simulink subsystem "Subsys_GFolConv_OuterCtrl_MatchCtrl"  (R2023b)
settings: Solver=VariableStepAuto  StartTime=0.0  StopTime=10.0  RelTol=1e-3
model mask{S_n=S_n, P_binst=P_binst, f_n=f_n, Q_ctrl_mode_m=Matching_Control_Q_ctrl_mode, T_PT1_Q_m=Matching_Control_T_PT1_Q, uq0ref_m=Matching_Control_QV_uq0ref, qmax_m=Matching_Control_QV_qmax, umax_m=Matching_Control_QV_umax, deadband_m=Matching_Control_QV_deadband, p_pu_m=Matching_Control_QP_P, q_pu_m=Matching_Control_QP_Q, p1_m=Matching_Control_QVDB_P1, p2_m=Matching_Control_QVDB_P2, p3_m=Matching_Control_QVDB_P3, p4_m=Matching_Control_QVDB_P4, cosphi_ref_m=Matching_Control_cosphi_ref, Q_direction_m=Matching_Control_cosphi_direction, T_s_ctrl=T_s_ctrl, datatype=datatype, K_matching=K_Matching_m, plant_ref=Plant_Ref, plant_model=Plant_Model, luenberger=Luenberger, Ts_matching=Ts_Matching_m}
  mask prompts: S_n "Nominal apparent power [VA]"; P_binst "Installed active power [W]"; f_n "Nominal frequency [Hz]"; Q_ctrl_mode_m "Q-control mode (1 = Q(V), 2 = Q(P), 3 = Q(V) with deadband, 4 = cosphi)"; T_PT1_Q_m "Time constant of reactive power PT1 delay [s]"; uq0ref_m "U_Q0ref [pu]"; qmax_m "|Q_max| [pu]"; umax_m "U_max [pu]"; deadband_m "Voltage deadband [+-%]"; p_pu_m "P_grid points [pu]"; q_pu_m "Q_grid points [pu]"; p1_m "P1 [V_grid, Q_grid] [pu]"; p2_m "P2 [V_grid, Q_grid] [pu]"; p3_m "P3 [V_grid, Q_grid] [pu]"; p4_m "P4 [V_grid, Q_grid] [pu]"; cosphi_ref_m "cos(phi)"; Q_direction_m "Reactive power flow direction (1 =ind. Q injection, 0 = ind. Q consumption)"; T_s_ctrl "Controller sample time [s]"; datatype "Signal data type"; K_matching "Gain Matching Control"; plant_ref "Reference model"; plant_model "Plant model"; luenberger "Luenberger observer"; Ts_matching "Time constant Matching Control"
undefined symbols (not defined in the file): DiscIntNeverNeededParam
libraries: simulink x5, spsSampleandHoldLib x2, cstblocks x2, dspswit3 x1
settings Model: Creator=j.jansen  LastModifiedBy=a.och
settings RTWCC: GPUComputeCapability=5.0

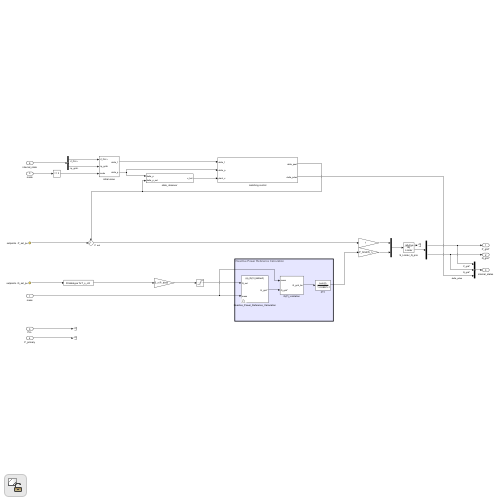
[thumbnail: Simulink's stored preview of the top-level diagram]
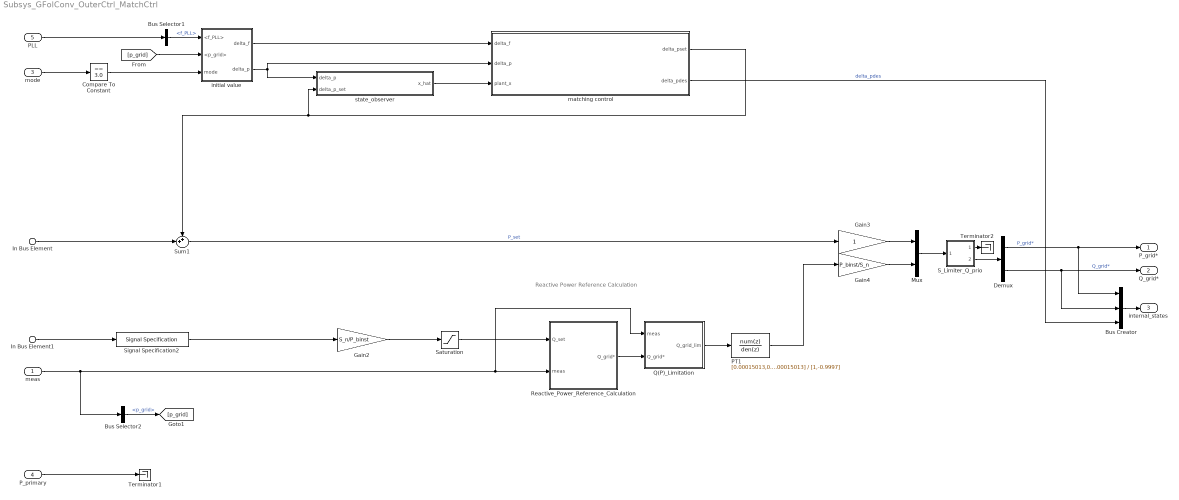
== system Subsys_GFolConv_OuterCtrl_MatchCtrl ==
  note: Reactive Power Reference Calculation
  meas : Inport
  In Bus Element : Inport  Port=2  PortName=setpoints  Element=P_set_pu
  In Bus Element1 : Inport  Port=2  PortName=setpoints  Element=Q_set_pu
  mode : Inport  Port=3
  P_primary : Inport  Port=4
  PLL : Inport  Port=5
  Bus Creator : BusCreator  Inputs=3
  Bus Selector1 : BusSelector  OutputSignals=f_PLL
  Bus Selector2 : BusSelector  OutputSignals=p_grid
  Compare To Constant : simulink/Logic and Bit Operations/Compare To Constant  relop===  const=3.0  OutDataTypeStr=boolean
  Demux : Demux  Outputs=2
  Gain2 : Gain  Gain=S_n/P_binst
  Gain3 : Gain
  Gain4 : Gain  Gain=P_binst/S_n
  Mux : Mux  Inputs=2
  PT1 : DiscreteFilter  Numerator=[0.00015013,0.00015013]  Denominator=[1,-0.9997]  SampleTime=T_s_ctrl
  Q(P)_Limitation : Subsystem
  Reactive_Power_Reference_Calculation : Subsystem  Variant=on
  S_Limiter_Q_prio : Subsystem  ReferencedSubsystem=dq_Limiter  X_dq_max=1  datatype=datatype
  Saturation : Saturate  UpperLimit=0.33  LowerLimit=-0.33
  Signal Specification2 : SignalSpecification  OutDataTypeStr=datatype  SampleTime=T_s_ctrl
  Sum1 : Sum  Inputs=++|
  Terminator1 : Terminator
  Terminator2 : Terminator
  initial value : Subsystem
  matching control : Subsystem
  state_observer : Subsystem
  P_grid* : Outport
  Q_grid* : Outport  Port=2
  internal_states : Outport  Port=3
  wires:
  Compare To Constant/1 -> initial value/3(mode)
  Gain2/1 -> Saturation/1
  Demux/1 -> P_grid*/1, Bus Creator/1  "P_grid*"
  Mux/1 -> S_Limiter_Q_prio/1
  S_Limiter_Q_prio/1 -> Terminator2/1
  Demux/2 -> Q_grid*/1, Bus Creator/2  "Q_grid*"
  Gain3/1 -> Mux/1
  Q(P)_Limitation/1(Q_grid_lim) -> PT1/1
  S_Limiter_Q_prio/2 -> Demux/1
  PT1/1 -> Gain4/1
  In Bus Element1/1 -> Signal Specification2/1
  Saturation/1 -> Reactive_Power_Reference_Calculation/1(Q_set)
  Reactive_Power_Reference_Calculation/1(Q_grid*) -> Q(P)_Limitation/2(Q_grid*)
  Gain4/1 -> Mux/2
  Signal Specification2/1 -> Gain2/1
  Bus Creator/1 -> internal_states/1
  state_observer/1(x_hat) -> matching control/3(plant_x)
  initial value/1("  delta_f ") -> matching control/1(delta_f)
  matching control/2(delta_pdes) -> Bus Creator/3  "delta_pdes"
  initial value/2("  delta_p") -> state_observer/1(delta_p), matching control/2(delta_p)
  matching control/1(delta_pset) -> state_observer/2(delta_p_set), Sum1/1
  In Bus Element/1 -> Sum1/2
  Sum1/1 -> Gain3/1  "P_set"
  mode/1 -> Compare To Constant/1
  meas/1 -> Reactive_Power_Reference_Calculation/2(meas), Q(P)_Limitation/1(meas), Bus Selector2/1
  P_primary/1 -> Terminator1/1
  PLL/1 -> Bus Selector1/1
  Bus Selector1/1 -> initial value/1(<f_PLL>)  "<f_PLL>"
  Bus Selector2/1 -> [p_grid]  "<p_grid>"
  [p_grid] -> initial value/2(<p_grid>)

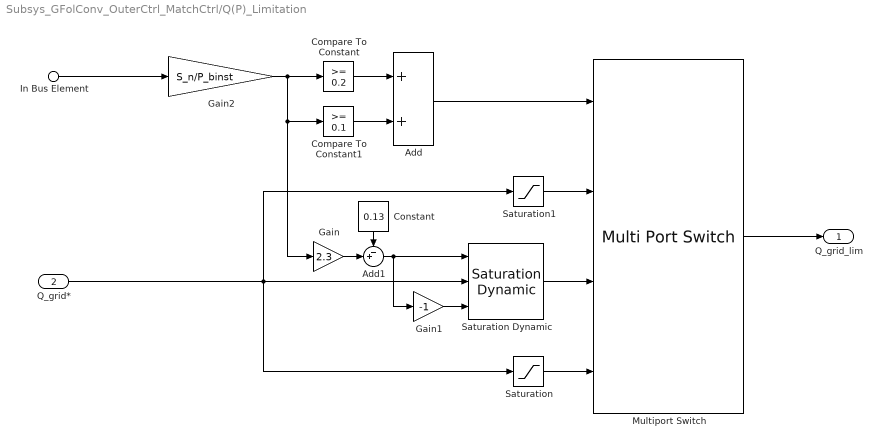
== system Subsys_GFolConv_OuterCtrl_MatchCtrl/Q(P)_Limitation ==
  In Bus Element : Inport  PortName=meas  Element=p_grid
  Q_grid* : Inport  Port=2
  Add : Sum
  Add1 : Sum  Inputs=-+|
  Compare To Constant : simulink/Logic and Bit Operations/Compare To Constant  relop=>=  const=0.2  OutDataTypeStr=uint8
  Compare To Constant1 : simulink/Logic and Bit Operations/Compare To Constant  relop=>=  const=0.1  OutDataTypeStr=uint8
  Constant : Constant  Value=0.13  OutDataTypeStr=datatype
  Gain : Gain  Gain=2.3
  Gain1 : Gain  Gain=-1
  Gain2 : Gain  Gain=S_n/P_binst
  Multiport Switch : MultiPortSwitch  DataPortOrder=Zero-based contiguous  zeroidx=on  SaturateOnIntegerOverflow=off  InputSameDT=off
  Saturation : Saturate  UpperLimit=0.33  LowerLimit=-0.33
  Saturation Dynamic : simulink/Discontinuities/Saturation Dynamic  OutMin=[]  OutMax=[]  OutDataTypeStr=Inherit: Same as second input  OutDataType=fixdt(1, 16)  OutScaling=2^-10  DoSatur=off
  Saturation1 : Saturate  UpperLimit=0.02  LowerLimit=-0.05
  Q_grid_lim : Outport
  wires:
  In Bus Element/1 -> Gain2/1
  Compare To Constant/1 -> Add/1
  Compare To Constant1/1 -> Add/2
  Add/1 -> Multiport Switch/1
  Saturation/1 -> Multiport Switch/4
  Saturation1/1 -> Multiport Switch/2
  Q_grid*/1 -> Saturation Dynamic/2, Saturation/1, Saturation1/1
  Multiport Switch/1 -> Q_grid_lim/1
  Saturation Dynamic/1 -> Multiport Switch/3
  Gain/1 -> Add1/2
  Constant/1 -> Add1/1
  Add1/1 -> Saturation Dynamic/1, Gain1/1
  Gain1/1 -> Saturation Dynamic/3
  Gain2/1 -> Gain/1, Compare To Constant1/1, Compare To Constant/1

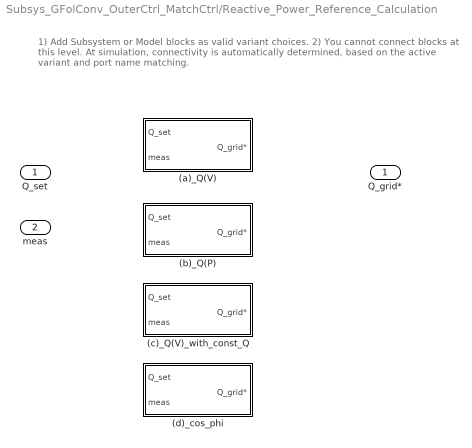
== system Subsys_GFolConv_OuterCtrl_MatchCtrl/Reactive_Power_Reference_Calculation ==
  note: 1) Add Subsystem or Model blocks as valid variant choices.
      | 2) You cannot connect blocks at this level. At simulation, connectivity is automatically
      | determined, based on the active variant and port name matching.
  Q_set : Inport
  meas : Inport  Port=2
  (a)_Q(V) : Subsystem  VariantControl=(default)
  (b)_Q(P) : Subsystem  VariantControl=Q_ctrl_mode_m == 2
  (c)_Q(V)_with_const_Q : Subsystem  VariantControl=Q_ctrl_mode_m == 3
  (d)_cos_phi : Subsystem  VariantControl=Q_ctrl_mode_m == 4
  Q_grid* : Outport

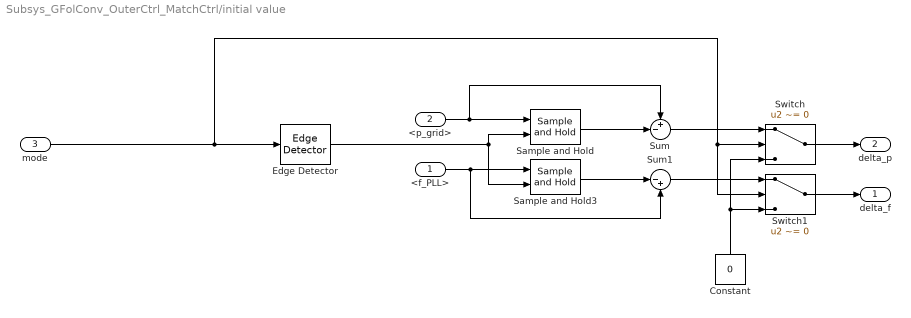
== system Subsys_GFolConv_OuterCtrl_MatchCtrl/initial value ==
  <f_PLL> : Inport
  <p_grid> : Inport  Port=2
  mode : Inport  Port=3
  Constant : Constant  Value=0  OutDataTypeStr=single
  Edge Detector : dspswit3/Edge Detector  InputProcessing=Columns as channels (frame based)
  Sample and Hold : spsSampleandHoldLib/Sample and Hold  ic=0  Ts=Ts_matching
      settings: LibrarySourceBlock=|
      | sps_lib/Control/Sample and
      | Hold
  Sample and Hold3 : spsSampleandHoldLib/Sample and Hold  ic=0  Ts=Ts_matching
      settings: LibrarySourceBlock=|
      | sps_lib/Control/Sample and
      | Hold
  Sum : Sum  Inputs=+-|
  Sum1 : Sum  Inputs=|-+
  Switch : Switch  Criteria=u2 ~= 0  SaturateOnIntegerOverflow=off  InputSameDT=off
  Switch1 : Switch  Criteria=u2 ~= 0  SaturateOnIntegerOverflow=off  InputSameDT=off
  "  delta_f " : Outport
  "  delta_p" : Outport  Port=2
  wires:
  Edge Detector/1 -> Sample and Hold/2, Sample and Hold3/2
  Constant/1 -> Switch/3, Switch1/3
  Switch1/1 -> "  delta_f "/1
  Switch/1 -> "  delta_p"/1
  Sum1/1 -> Switch1/1
  Sum/1 -> Switch/1
  Sample and Hold/1 -> Sum/2
  Sample and Hold3/1 -> Sum1/1
  mode/1 -> Switch1/2, Switch/2, Edge Detector/1
  <p_grid>/1 -> Sum/1, Sample and Hold/1
  <f_PLL>/1 -> Sample and Hold3/1, Sum1/2

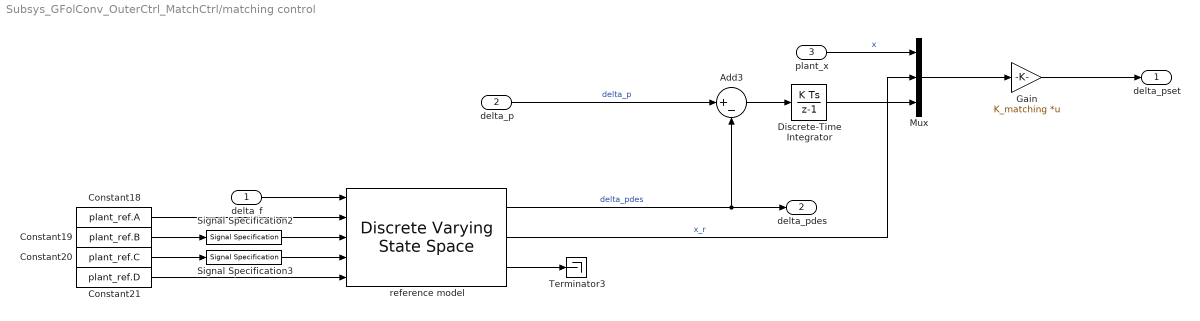
== system Subsys_GFolConv_OuterCtrl_MatchCtrl/matching control ==
  delta_f : Inport
  delta_p : Inport  Port=2
  plant_x : Inport  Port=3
  Add3 : Sum  Inputs=|+-
  Constant18 : Constant  Value=plant_ref.A  OutDataTypeStr=single  SampleTime=Ts_matching
  Constant19 : Constant  Value=plant_ref.B  OutDataTypeStr=single  SampleTime=Ts_matching
  Constant20 : Constant  Value=plant_ref.C  OutDataTypeStr=single  SampleTime=Ts_matching
  Constant21 : Constant  Value=plant_ref.D  OutDataTypeStr=single  SampleTime=Ts_matching
  Discrete-Time Integrator : DiscreteIntegrator  SampleTime=Ts_matching  ICPrevOutput=DiscIntNeverNeededParam  ICPrevScaledInput=DiscIntNeverNeededParam
  Gain : Gain  Gain=K_matching  Multiplication=Matrix(K*u)
  Mux : Mux  Inputs=3
  Signal Specification2 : SignalSpecification  Dimensions=[size(plant_ref.B,1), size(plant_ref.B,2)]  SampleTime=Ts_matching
  Signal Specification3 : SignalSpecification  Dimensions=[size(plant_ref.C,1), size(plant_ref.C,2)]  SampleTime=Ts_matching
  Terminator3 : Terminator
  reference model : cstblocks/Linear Parameter Varying/Discrete Varying State Space  x0=0  Ts=Ts_matching  OutputX=on  OutputDX=on  Feedthrough=on
  delta_pset : Outport
  delta_pdes : Outport  Port=2
  wires:
  Signal Specification3/1 -> reference model/4
  Signal Specification2/1 -> reference model/3
  Gain/1 -> delta_pset/1
  Mux/1 -> Gain/1
  Discrete-Time Integrator/1 -> Mux/3
  plant_x/1 -> Mux/1  "x"
  Add3/1 -> Discrete-Time Integrator/1
  reference model/1 -> Add3/2, delta_pdes/1  "delta_pdes"
  delta_p/1 -> Add3/1  "delta_p"
  reference model/3 -> Terminator3/1
  delta_f/1 -> reference model/1
  Constant18/1 -> reference model/2
  Constant20/1 -> Signal Specification3/1
  Constant21/1 -> reference model/5
  Constant19/1 -> Signal Specification2/1
  reference model/2 -> Mux/2  "x_r"

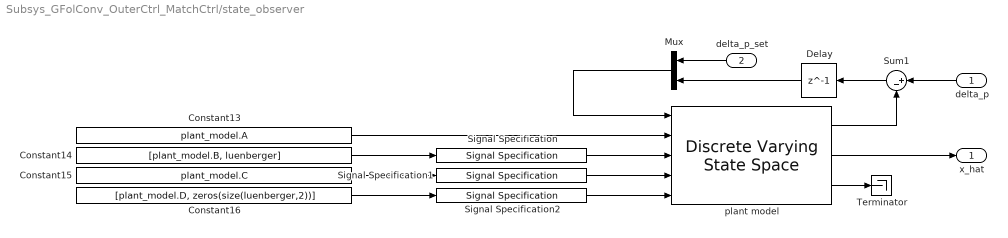
== system Subsys_GFolConv_OuterCtrl_MatchCtrl/state_observer ==
  delta_p : Inport
  delta_p_set : Inport  Port=2
  Constant13 : Constant  Value=plant_model.A  OutDataTypeStr=single  SampleTime=Ts_matching
  Constant14 : Constant  Value=[plant_model.B, luenberger]  OutDataTypeStr=single  SampleTime=Ts_matching
  Constant15 : Constant  Value=plant_model.C  OutDataTypeStr=single  SampleTime=Ts_matching
  Constant16 : Constant  Value=[plant_model.D, zeros(size(luenberger,2))]  OutDataTypeStr=single  SampleTime=Ts_matching
  Delay : Delay  DelayLength=1  SampleTime=Ts_matching
  Mux : Mux  Inputs=2
  Signal Specification : SignalSpecification  Dimensions=[size(plant_model.B,1),size(plant_model.B,2) + size(luenberger,2)]  SampleTime=Ts_matching
  Signal Specification1 : SignalSpecification  Dimensions=[size(plant_model.C,1),size(plant_model.C,2)]  SampleTime=Ts_matching
  Signal Specification2 : SignalSpecification  Dimensions=[size(plant_model.C,1),size(plant_model.B,2)+ size(luenberger,2)]  SampleTime=Ts_matching
  Sum1 : Sum  Inputs=|+-
  Terminator : Terminator
  plant model : cstblocks/Linear Parameter Varying/Discrete Varying State Space  x0=0  Ts=Ts_matching  OutputX=on  OutputDX=on  Feedthrough=on
  x_hat : Outport
  wires:
  plant model/3 -> Terminator/1
  delta_p_set/1 -> Mux/1
  Delay/1 -> Mux/2
  Signal Specification1/1 -> plant model/4
  Signal Specification/1 -> plant model/3
  delta_p/1 -> Sum1/1
  Constant16/1 -> Signal Specification2/1
  Constant14/1 -> Signal Specification/1
  Signal Specification2/1 -> plant model/5
  plant model/2 -> x_hat/1
  plant model/1 -> Sum1/2
  Constant15/1 -> Signal Specification1/1
  Sum1/1 -> Delay/1
  Mux/1 -> plant model/1
  Constant13/1 -> plant model/2

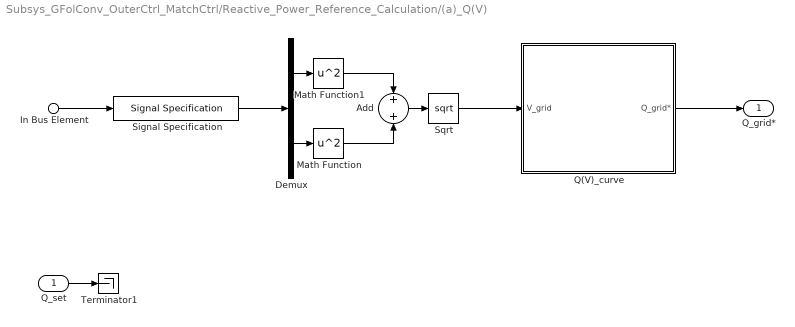
== system Subsys_GFolConv_OuterCtrl_MatchCtrl/Reactive_Power_Reference_Calculation/(a)_Q(V) ==
  Q_set : Inport
  In Bus Element : Inport  Port=2  PortName=meas  Element=dq+.v_grid_dq+
  Add : Sum  Inputs=+|+
  Demux : Demux  Outputs=2
  Math Function : Math  Operator=square
  Math Function1 : Math  Operator=square
  Q(V)_curve : Subsystem  mask{deadband=deadband_m, umax=umax_m, qmax=qmax_m, uq0ref=uq0ref_m}
      mask prompts: deadband "Voltage Deadband [+- %]"; umax "U_max [pu]"; qmax "|Q_max| [pu]"; uq0ref "U_Q0ref [pu]"
      mask DialogControl DescGroupVar Prompt: Q(V)-curve
      mask DialogControl DescTextVar Prompt: Q(V)-curve according to VDE 4110. Detailed parameter descriptions are given in the VDE 4110 document.
  Signal Specification : SignalSpecification  OutDataTypeStr=datatype  SampleTime=T_s_ctrl
  Sqrt : Sqrt
  Terminator1 : Terminator
  Q_grid* : Outport
  wires:
  In Bus Element/1 -> Signal Specification/1
  Q(V)_curve/1(Q_grid*) -> Q_grid*/1
  Demux/2 -> Math Function/1
  Demux/1 -> Math Function1/1
  Math Function1/1 -> Add/1
  Math Function/1 -> Add/2
  Add/1 -> Sqrt/1
  Sqrt/1 -> Q(V)_curve/1(V_grid)
  Q_set/1 -> Terminator1/1
  Signal Specification/1 -> Demux/1

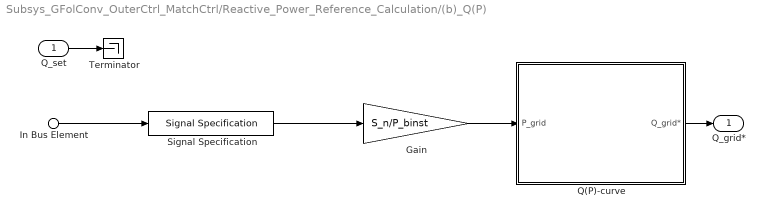
== system Subsys_GFolConv_OuterCtrl_MatchCtrl/Reactive_Power_Reference_Calculation/(b)_Q(P) ==
  Q_set : Inport
  In Bus Element : Inport  Port=2  PortName=meas  Element=p_grid
  Gain : Gain  Gain=S_n/P_binst
  Q(P)-curve : Subsystem  mask{q_pu=q_pu_m, p_pu=p_pu_m}
      mask prompts: q_pu "Q_grid points [pu]"; p_pu "P_grid points [pu]"
      mask DialogControl DescGroupVar Prompt: Q(P)-curve
      mask DialogControl DescTextVar Prompt: Q(P)-curve according to VDE 4110. Detailed parameter descriptions are given in the VDE 4110 document.
      mask DialogControl Control2 Prompt: In contrast to VDE 4110, here the active and reactive power values are given in active sign convention.
  Signal Specification : SignalSpecification  OutDataTypeStr=datatype  SampleTime=T_s_ctrl
  Terminator : Terminator
  Q_grid* : Outport
  wires:
  In Bus Element/1 -> Signal Specification/1
  Q_set/1 -> Terminator/1
  Q(P)-curve/1(Q_grid*) -> Q_grid*/1
  Gain/1 -> Q(P)-curve/1(P_grid)
  Signal Specification/1 -> Gain/1

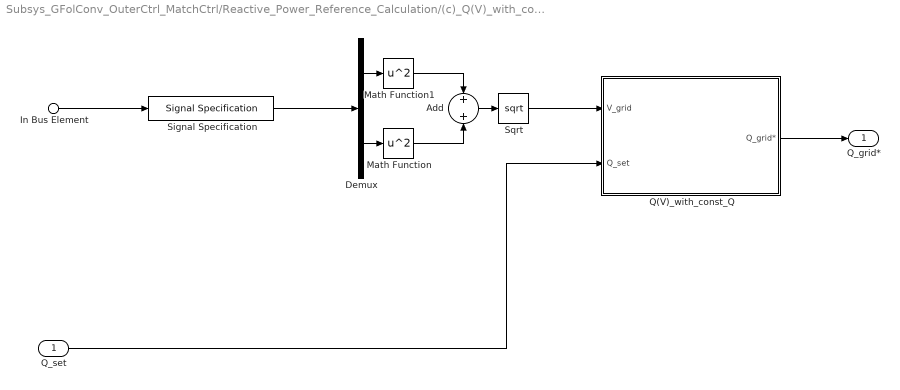
== system Subsys_GFolConv_OuterCtrl_MatchCtrl/Reactive_Power_Reference_Calculation/(c)_Q(V)_with_const_Q ==
  Q_set : Inport
  In Bus Element : Inport  Port=2  PortName=meas  Element=dq+.v_grid_dq+
  Add : Sum  Inputs=+|+
  Demux : Demux  Outputs=2
  Math Function : Math  Operator=square
  Math Function1 : Math  Operator=square
  Q(V)_with_const_Q : Subsystem  mask{p1=p1_m, p2=p2_m, p3=p3_m, p4=p4_m}
      mask prompts: p1 "P1 [V_grid, Q_grid] [pu]"; p2 "P2 [V_grid, Q_grid] [pu]"; p3 "P3 [V_grid, Q_grid] [pu]"; p4 "P4 [V_grid, Q_grid] [pu]"
      mask DialogControl DescGroupVar Prompt: Constant Q with voltage limitation
      mask DialogControl DescTextVar Prompt: Q(V)-curve according to VDE 4110. Detailed parameter descriptions are given in the VDE 4110 document.
      mask DialogControl Control2 Prompt: In contrast to VDE 4110, here the reactive power values are given in active sign convention.
  Signal Specification : SignalSpecification  OutDataTypeStr=datatype  SampleTime=T_s_ctrl
  Sqrt : Sqrt
  Q_grid* : Outport
  wires:
  In Bus Element/1 -> Signal Specification/1
  Q_set/1 -> Q(V)_with_const_Q/2(Q_set)
  Demux/1 -> Math Function1/1
  Add/1 -> Sqrt/1
  Math Function1/1 -> Add/1
  Math Function/1 -> Add/2
  Demux/2 -> Math Function/1
  Sqrt/1 -> Q(V)_with_const_Q/1(V_grid)
  Q(V)_with_const_Q/1(Q_grid*) -> Q_grid*/1
  Signal Specification/1 -> Demux/1

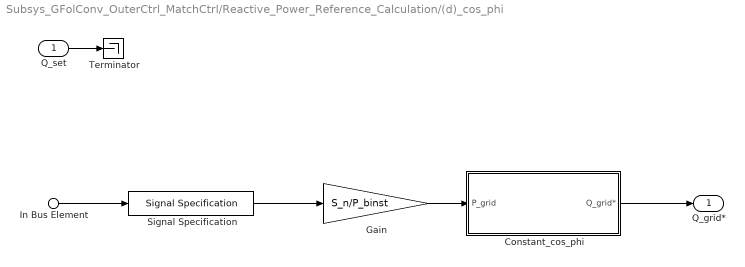
== system Subsys_GFolConv_OuterCtrl_MatchCtrl/Reactive_Power_Reference_Calculation/(d)_cos_phi ==
  Q_set : Inport
  In Bus Element : Inport  Port=2  PortName=meas  Element=p_grid
  Constant_cos_phi : Subsystem  mask{cosphi_ref=cosphi_ref_m, inductive_Q_infeed=Q_direction_m}
      mask prompts: cosphi_ref "cos(phi)"; inductive_Q_infeed "Reactive power flow direction (1 = ind. Q injection, 0 = ind. Q consumption)"
      mask DialogControl DescGroupVar Prompt: Constant cos(phi)
      mask DialogControl DescTextVar Prompt: Constant cos(phi) behavior according to VDE 4110. Detailed parameter descriptions are given in the VDE 4110 document.
  Gain : Gain  Gain=S_n/P_binst
  Signal Specification : SignalSpecification  OutDataTypeStr=datatype  SampleTime=T_s_ctrl
  Terminator : Terminator
  Q_grid* : Outport
  wires:
  In Bus Element/1 -> Signal Specification/1
  Q_set/1 -> Terminator/1
  Constant_cos_phi/1(Q_grid*) -> Q_grid*/1
  Gain/1 -> Constant_cos_phi/1(P_grid)
  Signal Specification/1 -> Gain/1

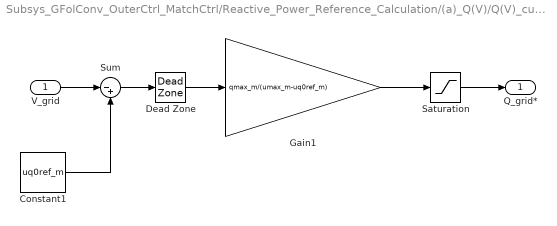
== system Subsys_GFolConv_OuterCtrl_MatchCtrl/Reactive_Power_Reference_Calculation/(a)_Q(V)/Q(V)_curve ==
  V_grid : Inport
  Constant1 : Constant  Value=uq0ref_m
  Dead Zone : DeadZone  LowerValue=-deadband/100  UpperValue=+deadband/100
  Gain1 : Gain  Gain=qmax_m/(umax_m-uq0ref_m)
  Saturation : Saturate  UpperLimit=qmax  LowerLimit=-qmax
  Sum : Sum  Inputs=|-+
  Q_grid* : Outport  VectorParamsAs1DForOutWhenUnconnected=off
  wires:
  V_grid/1 -> Sum/1
  Sum/1 -> Dead Zone/1
  Gain1/1 -> Saturation/1
  Dead Zone/1 -> Gain1/1
  Saturation/1 -> Q_grid*/1
  Constant1/1 -> Sum/2

== system Subsys_GFolConv_OuterCtrl_MatchCtrl/Reactive_Power_Reference_Calculation/(b)_Q(P)/Q(P)-curve ==
  P_grid : Inport
  1-D Lookup Table1 : Lookup_n-D  NumberOfTableDimensions=1  BreakpointsForDimension1=p_pu_m  Table=q_pu_m  InternalRulePriority=Speed  RndMeth=Simplest
  Q_grid* : Outport  VectorParamsAs1DForOutWhenUnconnected=off
  wires:
  P_grid/1 -> 1-D Lookup Table1/1
  1-D Lookup Table1/1 -> Q_grid*/1

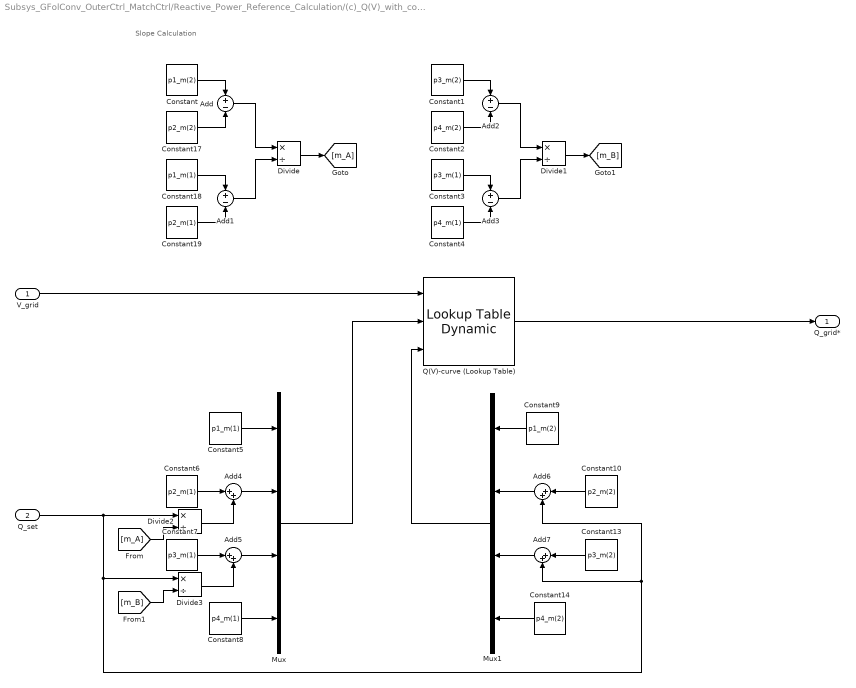
== system Subsys_GFolConv_OuterCtrl_MatchCtrl/Reactive_Power_Reference_Calculation/(c)_Q(V)_with_const_Q/Q(V)_with_const_Q ==
  note: Slope Calculation
  V_grid : Inport
  Q_set : Inport  Port=2
  Add{,1..3} (4 alike) : Sum  Inputs=+|-
  Add{4..7} (4 alike) : Sum  Inputs=|++
  Constant : Constant  Value=p1_m(2)
  Constant1 : Constant  Value=p3_m(2)
  Constant10 : Constant  Value=p2_m(2)
  Constant13 : Constant  Value=p3_m(2)
  Constant14 : Constant  Value=p4_m(2)
  Constant17 : Constant  Value=p2_m(2)
  Constant18 : Constant  Value=p1_m(1)
  Constant19 : Constant  Value=p2_m(1)
  Constant2 : Constant  Value=p4_m(2)
  Constant3 : Constant  Value=p3_m(1)
  Constant4 : Constant  Value=p4_m(1)
  Constant5 : Constant  Value=p1_m(1)
  Constant6 : Constant  Value=p2_m(1)
  Constant7 : Constant  Value=p3_m(1)
  Constant8 : Constant  Value=p4_m(1)
  Constant9 : Constant  Value=p1_m(2)
  Divide{,1..3} (4 alike) : Product  Inputs=*/
  Mux : Mux
  Mux1 : Mux
  Q(V)-curve (Lookup Table) : simulink/Lookup Tables/Lookup Table Dynamic  LookUpMeth=Interpolation-Use End Values  OutDataType=datatype  OutScaling=[]  OutputDataTypeScalingMode=Specify via dialog  OutDataTypeStr=datatype  DoSatur=off
  Q_grid* : Outport  VectorParamsAs1DForOutWhenUnconnected=off
  wires:
  V_grid/1 -> Q(V)-curve (Lookup Table)/1
  Q(V)-curve (Lookup Table)/1 -> Q_grid*/1
  Constant/1 -> Add/1
  Constant17/1 -> Add/2
  Constant19/1 -> Add1/2
  Constant18/1 -> Add1/1
  Add/1 -> Divide/1
  Add1/1 -> Divide/2
  Divide/1 -> [m_A]
  Divide1/1 -> [m_B]
  Constant3/1 -> Add3/1
  Add2/1 -> Divide1/1
  Constant4/1 -> Add3/2
  Add3/1 -> Divide1/2
  Constant2/1 -> Add2/2
  Constant1/1 -> Add2/1
  Constant5/1 -> Mux/1
  Constant8/1 -> Mux/4
  Mux/1 -> Q(V)-curve (Lookup Table)/2
  Mux1/1 -> Q(V)-curve (Lookup Table)/3
  Constant9/1 -> Mux1/1
  Constant14/1 -> Mux1/4
  Add5/1 -> Mux/3
  Add4/1 -> Mux/2
  Constant6/1 -> Add4/1
  Constant7/1 -> Add5/1
  Divide2/1 -> Add4/2
  Divide3/1 -> Add5/2
  [m_A] -> Divide2/2
  [m_B] -> Divide3/2
  Add6/1 -> Mux1/2
  Add7/1 -> Mux1/3
  Constant13/1 -> Add7/1
  Constant10/1 -> Add6/1
  Q_set/1 -> Add7/2, Add6/2, Divide3/1, Divide2/1

== system Subsys_GFolConv_OuterCtrl_MatchCtrl/Reactive_Power_Reference_Calculation/(d)_cos_phi/Constant_cos_phi ==
  P_grid : Inport
  Constant : Constant  Value=inductive_Q_infeed  OutDataTypeStr=datatype
  Gain1 : Gain  Gain=-1
  Gain2 : Gain  Gain=tan(acos(cosphi_ref_m))
  Switch : Switch  Criteria=u2 > Threshold  SaturateOnIntegerOverflow=off  InputSameDT=off
  Q_grid* : Outport  VectorParamsAs1DForOutWhenUnconnected=off
  wires:
  Gain2/1 -> Gain1/1, Switch/1
  P_grid/1 -> Gain2/1
  Constant/1 -> Switch/2
  Gain1/1 -> Switch/3
  Switch/1 -> Q_grid*/1
